simulink model "proj2"  (R2023a)
settings: Solver=VariableStepAuto  StartTime=0.0  StopTime=10.0  RelTol=1e-3
settings Model: Creator=Mariam Soliman  LastModifiedBy=Mariam Soliman

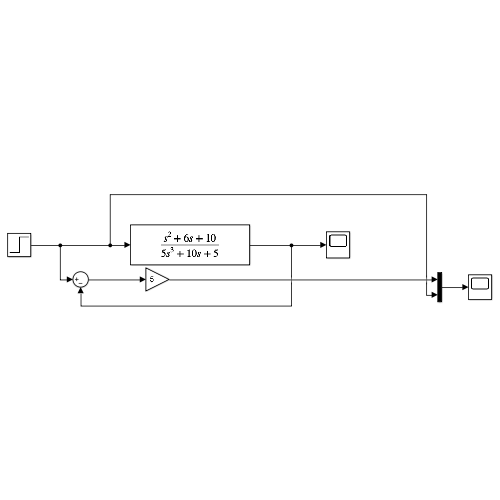
[thumbnail: Simulink's stored preview of the top-level diagram]
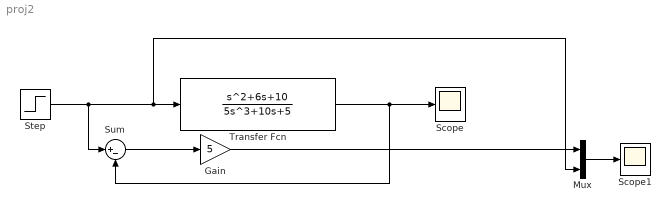
== system proj2 ==
  Gain : Gain  Gain=5
  Mux : Mux  Inputs=2
  Scope : Scope
  Scope1 : Scope
  Step : Step  SampleTime=0
  Sum : Sum  Inputs=|+-
  Transfer Fcn : TransferFcn  Numerator=[1 6 10]  Denominator="[5  0 10  5]"  ParameterTunability=Unconstrained
  wires:
  Transfer Fcn/1 -> Sum/2, Scope/1
  Step/1 -> Sum/1, Mux/2, Transfer Fcn/1
  Sum/1 -> Gain/1
  Gain/1 -> Mux/1
  Mux/1 -> Scope1/1
